simulink model "flight_simulation_6dof"  (R2025b)
settings: Solver=ode4  StartTime=0.0  StopTime=8.6  FixedStep=1/1000  RelTol=1e-3  AbsTol=1e-3  EnableMultiTasking=on
undefined symbols (not defined in the file): X, Y, Z
libraries: nesl_utility x122, sm_lib x98, simulink_extras x48, aerolibatmos2 x4, sharedtransform x4
(part 5 of 6)

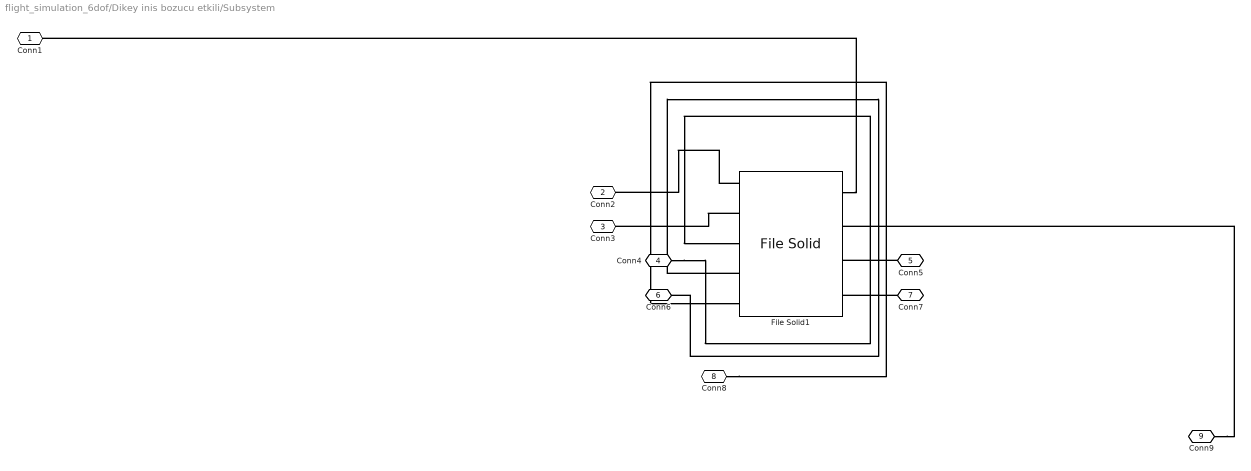
== system flight_simulation_6dof/Dikey inis bozucu etkili/Subsystem ==
  File Solid1 : sm_lib/Body Elements/File Solid  ExtGeomFileName=Roket 2926 Montaj Koordinat Merkeze Alınmış.STEP  UnitType=FromFile  ExtGeomFileUnits=m  StepReaderType=HEX  ExportConvexHullGeometry=off  InertiaType=Custom  BasedOnType=Mass  Density=1000  DensityUnits=kg/m^3  Mass=25  MassUnits=kg  CenterOfMass=[0 0 0.367]  CenterOfMassUnits=m  MomentsOfInertia=[3.842 3.842 1.406]  MomentsOfInertiaUnits=kg*m^2  ProductsOfInertia=[0 0 0]  ProductsOfInertiaUnits=kg*m^2  GraphicType=FromGeometry  MarkerShape=Sphere  MarkerSize=10  GraphicVisPropType=SimpleVisualProperties  GraphicDiffuseColor=[0.5 0.5 0.5]  GraphicOpacity=1  GraphicSpecularColor=[0.5 0.5 0.5 1.0]  GraphicAmbientColor=[0.15 0.15 0.15 1.0]  GraphicEmissiveColor=[0.0 0.0 0.0 1.0]  GraphicShininess=75  DoExposeReferenceFrame=on  SerializedFrames=|
      | <Frames>
      | 
      |   <Frame>
      |     <Id>Frame1</Id>
      |     <Value>
      |       <Name>Nozzle Frame</Name>
      |       <Origin>
      |         <Source>GeometricFeature</Source>
      |         <FeatureName>planar surface 207</FeatureName>
      |       </Origin>
      |       <PrimaryAxis>
      |         <DefinedDirection>+Z</DefinedDirection>
      |         <Source>ReferenceFrame</Source>
      |         <SourceDirection>+Z</SourceDirection>
      |         <FeatureName></FeatureName>
      |       </PrimaryAxis>
      |       <SecondaryAxis>
      |         <DefinedDirection>+X</DefinedDirection>
      |         <Source>ReferenceFrame</Source>
      |         <SourceDirection>+X</SourceDirection>
      |         <FeatureName></FeatureName>
      |       </SecondaryAxis>
      |     </Value>
      |   </Frame>
      | 
      |   <Frame>
      |     <Id>Frame3</Id>
      |     <Value>
      |       <Name>FN</Name>
      |       <Origin>
      |         <Source>GeometricFeature</Source>
      |         <FeatureName>planar surface 225</FeatureName>
      |       </Origin>
      |       <PrimaryAxis>
      |         <DefinedDirection>+Z</DefinedDirection>
      |         <Source>ReferenceFrame</Source>
      |         <SourceDirection>+X</SourceDirection>
      |         <FeatureName></FeatureName>
      |       </PrimaryAxis>
      |       <SecondaryAxis>
      |         <DefinedDirection>+X</DefinedDirection>
      |         <Source>ReferenceFrame</Source>
      |         <SourceDirection>-Z</SourceDirection>
      |         <FeatureName></FeatureName>
      |       </SecondaryAxis>
      |     </Value>
      |   </Frame>
      | 
      |   <Frame>
      |     <Id>Frame2</Id>
      |     <Value>
      |       <Name>Ref_Gas_Container</Name>
      |       <Origin>
      |         <Source>GeometricFeature</Source>
      |         <FeatureName>circular curve 1254</FeatureName>
      |       </Origin>
      |       <PrimaryAxis>
      |         <DefinedDirection>+Z</DefinedDirection>
      |         <Source>ReferenceFrame</Source>
      |         <SourceDirection>+Z</SourceDirection>
      |         <FeatureName></FeatureName>
      |       </PrimaryAxis>
      |       <SecondaryAxis>
      |         <DefinedDirection>+X</DefinedDirection>
      |         <Source>ReferenceFrame</Source>
      |         <SourceDirection>+X</SourceDirection>
      |         <FeatureName></FeatureName>
      |       </SecondaryAxis>
      |     </Value>
      |   </Frame>
      | 
      |   <Frame>
      |     <Id>Frame4</Id>
      |     <Value>
      |       <Name>LL1</Name>
      |       <Origin>
      |         <Source>GeometricFeature</Source>
      |         <FeatureName>circular curve 1452</FeatureName>
      |       </Origin>
      |       <PrimaryAxis>
      |         <DefinedDirection>+Z</DefinedDirection>
      |         <Source>ReferenceFrame</Source>
      |         <SourceDirection>+Z</SourceDirection>
      |         <FeatureName></FeatureName>
      |       </PrimaryAxis>
      |       <SecondaryAxis>
      |         <DefinedDirection>+X</DefinedDirection>
      |         <Source>ReferenceFrame</Source>
      |         <SourceDirection>+X</SourceDirection>
      |         <FeatureName></FeatureName>
      |       </SecondaryAxis>
      |     </Value>
      |   </Frame>
      | 
      |   <Frame>
      |     <Id>Frame5</Id>
      |     <Value>
      |       <Name>LL2</Name>
      |       <Origin>
      |         <Source>GeometricFeature</Source>
      |         <FeatureName>circular curve 188</FeatureName>
      |       </Origin>
      |       <PrimaryAxis>
      |         <DefinedDirection>+Z</DefinedDirection>
      |         <Source>ReferenceFrame</Source>
      |         <SourceDirection>+Z</SourceDirection>
      |         <FeatureName></FeatureName>
      |       </PrimaryAxis>
      |       <SecondaryAxis>
      |         <DefinedDirection>+X</DefinedDirection>
      |         <Source>ReferenceFrame</Source>
      |         <SourceDirection>+X</SourceDirection>
      |         <FeatureName></FeatureName>
      |       </SecondaryAxis>
      |     </Value>
      |   </Frame>
      | 
      |   <Frame>
      |     <Id>Frame6</Id>
      |     <Value>
      |       <Name>LL3</Name>
      |       <Origin>
      |         <Source>GeometricFeature</Source>
      |         <FeatureName>circular curve 1193</FeatureName>
      |       </Origin>
      |       <PrimaryAxis>
      |         <DefinedDirection>+Z</DefinedDirection>
      |         <Source>ReferenceFrame</Source>
      |         <SourceDirection>+Z</SourceDirection>
      |         <FeatureName></FeatureName>
      |       </PrimaryAxis>
      |       <SecondaryAxis>
      |         <DefinedDirection>+X</DefinedDirection>
      |         <Source>ReferenceFrame</Source>
      |         <SourceDirection>+X</SourceDirection>
      |         <FeatureName></FeatureName>
      |       </SecondaryAxis>
      |     </Value>
      |   </Frame>
      | 
      |   <Frame>
      |     <Id>Frame7</Id>
      |     <Value>
      |       <Name>LL4</Name>
      |       <Origin>
      |         <Source>GeometricFeature</Source>
      |         <FeatureName>circular curve 1537</FeatureName>
      |       </Origin>
      |       <PrimaryAxis>
      |         <DefinedDirection>+Z</DefinedDirection>
      |         <Source>ReferenceFrame</Source>
      |         <SourceDirection>+Z</SourceDirection>
      |         <FeatureName></FeatureName>
      |       </PrimaryAxis>
      |       <SecondaryAxis>
      |         <DefinedDirection>+X</DefinedDirection>
      |         <Source>ReferenceFrame</Source>
      |         <SourceDirection>+X</SourceDirection>
      |         <FeatureName></FeatureName>
      |       </SecondaryAxis>
      |     </Value>
      |   </Frame>
      | 
      |   <Frame>
      |     <Id>Frame8</Id>
      |     <Value>
      |       <Name>Dış Kuvvet</Name>
      |       <Origin>
      |         <Source>GeometricFeature</Source>
      |         <FeatureName>cylindrical surface 168</FeatureName>
      |       </Origin>
      |       <PrimaryAxis>
      |         <DefinedDirection>+Z</DefinedDirection>
      |         <Source>ReferenceFrame</Source>
      |         <SourceDirection>+Z</SourceDirection>
      |         <FeatureName></FeatureName>
      |       </PrimaryAxis>
      |       <SecondaryAxis>
      |         <DefinedDirection>+X</DefinedDirection>
      |         <Source>ReferenceFrame</Source>
      |         <SourceDirection>-X</SourceDirection>
      |         <FeatureName></FeatureName>
      |       </SecondaryAxis>
      |     </Value>
      |   </Frame>
      | 
      | </Frames>
  Conn1 : PMIOPort  Side=Right
  Conn2 : PMIOPort  Port=2  Side=Left
  Conn3 : PMIOPort  Port=3  Side=Left
  Conn4 : PMIOPort  Port=4  Side=Left
  Conn5 : PMIOPort  Port=5  Side=Right
  Conn6 : PMIOPort  Port=6  Side=Left
  Conn7 : PMIOPort  Port=7  Side=Right
  Conn8 : PMIOPort  Port=8  Side=Left
  Conn9 : PMIOPort  Port=9  Side=Right
  connections:
  Conn4/RConn1 -- File Solid1/LConn3
  File Solid1/LConn2 -- Conn3/RConn1
  File Solid1/LConn1 -- Conn2/RConn1
  Conn9/RConn1 -- File Solid1/RConn2
  Conn8/RConn1 -- File Solid1/LConn5
  File Solid1/LConn4 -- Conn6/RConn1
  File Solid1/RConn1 -- Conn1/RConn1
  Conn7/RConn1 -- File Solid1/RConn4
  Conn5/RConn1 -- File Solid1/RConn3

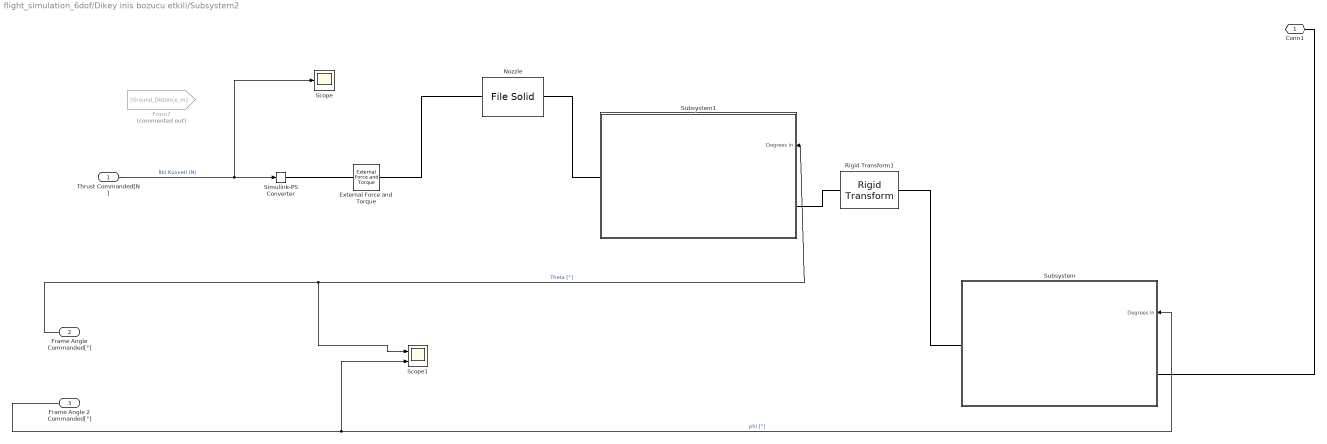
== system flight_simulation_6dof/Dikey inis bozucu etkili/Subsystem2 ==
  Thrust Commanded[N] : Inport
  Frame Angle Commanded[°] : Inport  Port=2
  Frame Angle 2 Commanded[°] : Inport  Port=3
  External Force and Torque : sm_lib/Forces and Torques/External Force and Torque  EnableForceX=off  EnableForceY=off  EnableForceZ=on  EnableForce=off  ForceResolutionFrame=AttachedFrame  EnableTorqueX=off  EnableTorqueY=off  EnableTorqueZ=off  EnableTorque=off  TorqueResolutionFrame=AttachedFrame
  From7 : From  Commented=on  GotoTag=Ground_Distance_m
  Nozzle : sm_lib/Body Elements/File Solid  ExtGeomFileName=C:\Users\HASAN BARAN\Desktop\ucusbenzetimson\S-TEK STEP DOSYALAR\nozzle.STEP  UnitType=FromFile  ExtGeomFileUnits=m  StepReaderType=HEX  ExportConvexHullGeometry=off  InertiaType=Custom  BasedOnType=DensityFromFile  Density=1000  DensityUnits=kg/m^3  Mass=1  MassUnits=kg  CenterOfMass=[0 0 0]  CenterOfMassUnits=m  MomentsOfInertia=[1 1 1]  MomentsOfInertiaUnits=kg*m^2  ProductsOfInertia=[0 0 0]  ProductsOfInertiaUnits=kg*m^2  GraphicType=FromGeometry  MarkerShape=Sphere  MarkerSize=10  GraphicVisPropType=SimpleVisualProperties  GraphicDiffuseColor=[0.5 0.5 0.5]  GraphicOpacity=1  GraphicSpecularColor=[0.5 0.5 0.5 1.0]  GraphicAmbientColor=[0.15 0.15 0.15 1.0]  GraphicEmissiveColor=[0.0 0.0 0.0 1.0]  GraphicShininess=75  DoExposeReferenceFrame=off  SerializedFrames=|
      | <Frames>
      | 
      |   <Frame>
      |     <Id>Frame1</Id>
      |     <Value>
      |       <Name>NF</Name>
      |       <Origin>
      |         <Source>GeometricFeature</Source>
      |         <FeatureName>circular curve 24</FeatureName>
      |       </Origin>
      |       <PrimaryAxis>
      |         <DefinedDirection>+Z</DefinedDirection>
      |         <Source>ReferenceFrame</Source>
      |         <SourceDirection>+X</SourceDirection>
      |         <FeatureName></FeatureName>
      |       </PrimaryAxis>
      |       <SecondaryAxis>
      |         <DefinedDirection>+X</DefinedDirection>
      |         <Source>ReferenceFrame</Source>
      |         <SourceDirection>-Z</SourceDirection>
      |         <FeatureName></FeatureName>
      |       </SecondaryAxis>
      |     </Value>
      |   </Frame>
      | 
      |   <Frame>
      |     <Id>Frame2</Id>
      |     <Value>
      |       <Name>Thrust</Name>
      |       <Origin>
      |         <Source>GeometricFeature</Source>
      |         <FeatureName>planar surface 3</FeatureName>
      |       </Origin>
      |       <PrimaryAxis>
      |         <DefinedDirection>+Z</DefinedDirection>
      |         <Source>ReferenceFrame</Source>
      |         <SourceDirection>+Z</SourceDirection>
      |         <FeatureName></FeatureName>
      |       </PrimaryAxis>
      |       <SecondaryAxis>
      |         <DefinedDirection>+X</DefinedDirection>
      |         <Source>ReferenceFrame</Source>
      |         <SourceDirection>+X</SourceDirection>
      |         <FeatureName></FeatureName>
      |       </SecondaryAxis>
      |     </Value>
      |   </Frame>
      | 
      | </Frames>
  Rigid Transform1 : sm_lib/Frames and Transforms/Rigid Transform  RotationMethod=StandardAxis  FollAlignAxisA=+X  BaseAlignAxisA=+Y  FollAlignAxisB=+Y  BaseAlignAxisB=+Z  RotationStandardAxis=+X  RotationAngle=-90  RotationAngleUnits=deg  RotationArbitraryAxis=[0 0 1]  RotationSequenceAxes=FollowerAxes  RotationSequence=XYX  RotationSequenceAngles=[0 0 0]  RotationSequenceAnglesUnits=deg  RotationMatrix=[1 0 0;0 1 0;0 0 1]  Quaternion=[1 0 0 0]  TranslationMethod=None  TranslationCartesianOffset=[0 0 0]  TranslationCartesianOffsetUnits=m  TranslationStandardAxis=+X  TranslationStandardOffset=0  TranslationStandardOffsetUnits=m  TranslationROffset=0  TranslationROffsetUnits=m  TranslationThetaOffset=0  TranslationThetaOffsetUnits=deg  TranslationZOffset=0  TranslationZOffsetUnits=m
  Scope : Scope
      settings: ActiveDisplayYMinimum=-11.060688029355445  ActiveDisplayYMaximum=24.029985729120519  DataLoggingVariableName=ScopeData6
  Scope1 : Scope  NumInputPorts=2
      settings: ActiveDisplayYMinimum=-79.822032700952221  ActiveDisplayYMaximum=168.51424627565183  DataLoggingVariableName=ScopeData15
  Simulink-PS Converter : nesl_utility/Simulink-PS Converter  PhysicalDomain=network_engine_domain  SubClassName=ps_input  LeftPortType=input  RightPortType=output  PseudoPeriodic=off  Frequencies=[]  NoiseDistribution=none  NoiseParameters=[]  Unit=1  AffineConversion=off  FilteringAndDerivatives=provide  SimscapeFilterOrder=1  InputFilterTimeConstant=0.001  UdotUserProvided=0
  Subsystem : Subsystem
  Subsystem1 : Subsystem
  Conn1 : PMIOPort  Side=Right
  wires:
  Frame Angle 2 Commanded[°]/1 -> Subsystem/1(Degrees in), Scope1/2  "phi [°]"
  Frame Angle Commanded[°]/1 -> Scope1/1, Subsystem1/1(Degrees in)  "Theta [°]"
  Thrust Commanded[N]/1 -> Simulink-PS Converter/1, Scope/1  "İtki Kuvveti (N)"
  connections:
  Simulink-PS Converter/RConn1 -- External Force and Torque/LConn1
  Subsystem/LConn1 -- Conn1/RConn1
  Subsystem/RConn1 -- Rigid Transform1/LConn1
  Rigid Transform1/RConn1 -- Subsystem1/LConn1
  External Force and Torque/RConn1 -- Nozzle/RConn1
  Subsystem1/RConn1 -- Nozzle/LConn1

== system flight_simulation_6dof/Yerden kalkis/MassModel1 ==
  Maximum Mass of Gas [kg] : Constant  Value=5
  Scope : Scope
      settings: ActiveDisplayYMinimum=-0.62488749999999993  ActiveDisplayYMaximum=5.6249875  DataLoggingVariableName=ScopeData11
  m_int : Integrator  InitialConditionSource=external  InitialCondition=31  LimitOutput=on  UpperSaturationLimit=5  LowerSaturationLimit=0.0001
  mdot_cmd : Constant  Commented=on  Value=0.9
  mdot_cmd2 : Step  Time=1.1  After=0.9  SampleTime=0
  negate : Gain  Gain=-1
  Mass of Gas [kg] : Outport
  wires:
  mdot_cmd2/1 -> negate/1
  negate/1 -> m_int/1
  m_int/1 -> Scope/1, Mass of Gas [kg]/1
  Maximum Mass of Gas [kg]/1 -> m_int/2

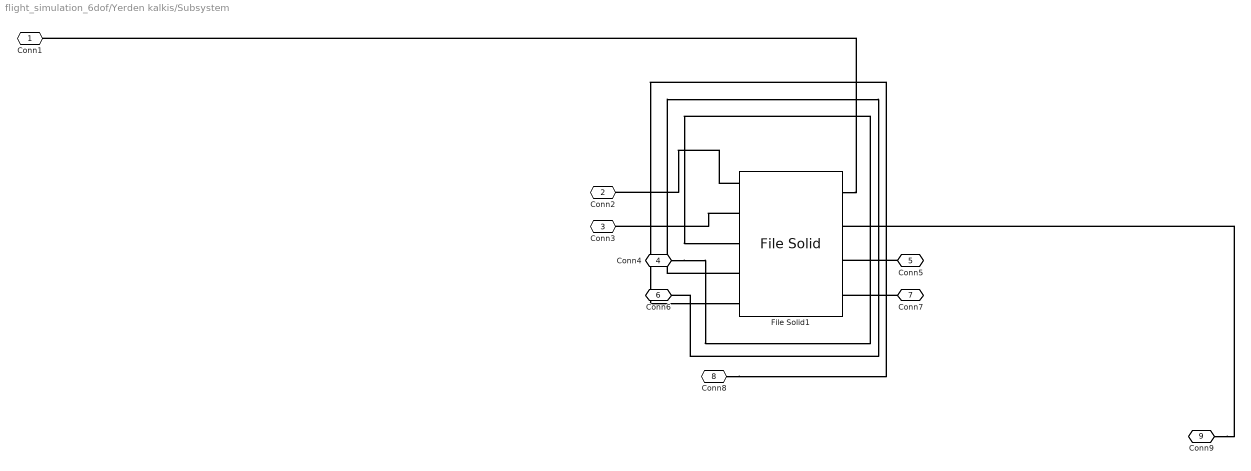
== system flight_simulation_6dof/Yerden kalkis/Subsystem ==
  File Solid1 : sm_lib/Body Elements/File Solid  ExtGeomFileName=Roket 2926 Montaj Koordinat Merkeze Alınmış.STEP  UnitType=FromFile  ExtGeomFileUnits=m  StepReaderType=HEX  ExportConvexHullGeometry=off  InertiaType=Custom  BasedOnType=Mass  Density=1000  DensityUnits=kg/m^3  Mass=25  MassUnits=kg  CenterOfMass=[0 0 0.367]  CenterOfMassUnits=m  MomentsOfInertia=[3.842 3.842 1.406]  MomentsOfInertiaUnits=kg*m^2  ProductsOfInertia=[0 0 0]  ProductsOfInertiaUnits=kg*m^2  GraphicType=FromGeometry  MarkerShape=Sphere  MarkerSize=10  GraphicVisPropType=SimpleVisualProperties  GraphicDiffuseColor=[0.5 0.5 0.5]  GraphicOpacity=1  GraphicSpecularColor=[0.5 0.5 0.5 1.0]  GraphicAmbientColor=[0.15 0.15 0.15 1.0]  GraphicEmissiveColor=[0.0 0.0 0.0 1.0]  GraphicShininess=75  DoExposeReferenceFrame=on  SerializedFrames=|
      | <Frames>
      | 
      |   <Frame>
      |     <Id>Frame1</Id>
      |     <Value>
      |       <Name>Nozzle Frame</Name>
      |       <Origin>
      |         <Source>GeometricFeature</Source>
      |         <FeatureName>planar surface 207</FeatureName>
      |       </Origin>
      |       <PrimaryAxis>
      |         <DefinedDirection>+Z</DefinedDirection>
      |         <Source>ReferenceFrame</Source>
      |         <SourceDirection>+Z</SourceDirection>
      |         <FeatureName></FeatureName>
      |       </PrimaryAxis>
      |       <SecondaryAxis>
      |         <DefinedDirection>+X</DefinedDirection>
      |         <Source>ReferenceFrame</Source>
      |         <SourceDirection>+X</SourceDirection>
      |         <FeatureName></FeatureName>
      |       </SecondaryAxis>
      |     </Value>
      |   </Frame>
      | 
      |   <Frame>
      |     <Id>Frame3</Id>
      |     <Value>
      |       <Name>FN</Name>
      |       <Origin>
      |         <Source>GeometricFeature</Source>
      |         <FeatureName>planar surface 225</FeatureName>
      |       </Origin>
      |       <PrimaryAxis>
      |         <DefinedDirection>+Z</DefinedDirection>
      |         <Source>ReferenceFrame</Source>
      |         <SourceDirection>+X</SourceDirection>
      |         <FeatureName></FeatureName>
      |       </PrimaryAxis>
      |       <SecondaryAxis>
      |         <DefinedDirection>+X</DefinedDirection>
      |         <Source>ReferenceFrame</Source>
      |         <SourceDirection>-Z</SourceDirection>
      |         <FeatureName></FeatureName>
      |       </SecondaryAxis>
      |     </Value>
      |   </Frame>
      | 
      |   <Frame>
      |     <Id>Frame2</Id>
      |     <Value>
      |       <Name>Ref_Gas_Container</Name>
      |       <Origin>
      |         <Source>GeometricFeature</Source>
      |         <FeatureName>circular curve 1254</FeatureName>
      |       </Origin>
      |       <PrimaryAxis>
      |         <DefinedDirection>+Z</DefinedDirection>
      |         <Source>ReferenceFrame</Source>
      |         <SourceDirection>+Z</SourceDirection>
      |         <FeatureName></FeatureName>
      |       </PrimaryAxis>
      |       <SecondaryAxis>
      |         <DefinedDirection>+X</DefinedDirection>
      |         <Source>ReferenceFrame</Source>
      |         <SourceDirection>+X</SourceDirection>
      |         <FeatureName></FeatureName>
      |       </SecondaryAxis>
      |     </Value>
      |   </Frame>
      | 
      |   <Frame>
      |     <Id>Frame4</Id>
      |     <Value>
      |       <Name>LL1</Name>
      |       <Origin>
      |         <Source>GeometricFeature</Source>
      |         <FeatureName>circular curve 1452</FeatureName>
      |       </Origin>
      |       <PrimaryAxis>
      |         <DefinedDirection>+Z</DefinedDirection>
      |         <Source>ReferenceFrame</Source>
      |         <SourceDirection>+Z</SourceDirection>
      |         <FeatureName></FeatureName>
      |       </PrimaryAxis>
      |       <SecondaryAxis>
      |         <DefinedDirection>+X</DefinedDirection>
      |         <Source>ReferenceFrame</Source>
      |         <SourceDirection>+X</SourceDirection>
      |         <FeatureName></FeatureName>
      |       </SecondaryAxis>
      |     </Value>
      |   </Frame>
      | 
      |   <Frame>
      |     <Id>Frame5</Id>
      |     <Value>
      |       <Name>LL2</Name>
      |       <Origin>
      |         <Source>GeometricFeature</Source>
      |         <FeatureName>circular curve 188</FeatureName>
      |       </Origin>
      |       <PrimaryAxis>
      |         <DefinedDirection>+Z</DefinedDirection>
      |         <Source>ReferenceFrame</Source>
      |         <SourceDirection>+Z</SourceDirection>
      |         <FeatureName></FeatureName>
      |       </PrimaryAxis>
      |       <SecondaryAxis>
      |         <DefinedDirection>+X</DefinedDirection>
      |         <Source>ReferenceFrame</Source>
      |         <SourceDirection>+X</SourceDirection>
      |         <FeatureName></FeatureName>
      |       </SecondaryAxis>
      |     </Value>
      |   </Frame>
      | 
      |   <Frame>
      |     <Id>Frame6</Id>
      |     <Value>
      |       <Name>LL3</Name>
      |       <Origin>
      |         <Source>GeometricFeature</Source>
      |         <FeatureName>circular curve 1193</FeatureName>
      |       </Origin>
      |       <PrimaryAxis>
      |         <DefinedDirection>+Z</DefinedDirection>
      |         <Source>ReferenceFrame</Source>
      |         <SourceDirection>+Z</SourceDirection>
      |         <FeatureName></FeatureName>
      |       </PrimaryAxis>
      |       <SecondaryAxis>
      |         <DefinedDirection>+X</DefinedDirection>
      |         <Source>ReferenceFrame</Source>
      |         <SourceDirection>+X</SourceDirection>
      |         <FeatureName></FeatureName>
      |       </SecondaryAxis>
      |     </Value>
      |   </Frame>
      | 
      |   <Frame>
      |     <Id>Frame7</Id>
      |     <Value>
      |       <Name>LL4</Name>
      |       <Origin>
      |         <Source>GeometricFeature</Source>
      |         <FeatureName>circular curve 1537</FeatureName>
      |       </Origin>
      |       <PrimaryAxis>
      |         <DefinedDirection>+Z</DefinedDirection>
      |         <Source>ReferenceFrame</Source>
      |         <SourceDirection>+Z</SourceDirection>
      |         <FeatureName></FeatureName>
      |       </PrimaryAxis>
      |       <SecondaryAxis>
      |         <DefinedDirection>+X</DefinedDirection>
      |         <Source>ReferenceFrame</Source>
      |         <SourceDirection>+X</SourceDirection>
      |         <FeatureName></FeatureName>
      |       </SecondaryAxis>
      |     </Value>
      |   </Frame>
      | 
      |   <Frame>
      |     <Id>Frame8</Id>
      |     <Value>
      |       <Name>Dış Kuvvet</Name>
      |       <Origin>
      |         <Source>GeometricFeature</Source>
      |         <FeatureName>cylindrical surface 168</FeatureName>
      |       </Origin>
      |       <PrimaryAxis>
      |         <DefinedDirection>+Z</DefinedDirection>
      |         <Source>ReferenceFrame</Source>
      |         <SourceDirection>+Z</SourceDirection>
      |         <FeatureName></FeatureName>
      |       </PrimaryAxis>
      |       <SecondaryAxis>
      |         <DefinedDirection>+X</DefinedDirection>
      |         <Source>ReferenceFrame</Source>
      |         <SourceDirection>-X</SourceDirection>
      |         <FeatureName></FeatureName>
      |       </SecondaryAxis>
      |     </Value>
      |   </Frame>
      | 
      | </Frames>
  Conn1 : PMIOPort  Side=Right
  Conn2 : PMIOPort  Port=2  Side=Left
  Conn3 : PMIOPort  Port=3  Side=Left
  Conn4 : PMIOPort  Port=4  Side=Left
  Conn5 : PMIOPort  Port=5  Side=Right
  Conn6 : PMIOPort  Port=6  Side=Left
  Conn7 : PMIOPort  Port=7  Side=Right
  Conn8 : PMIOPort  Port=8  Side=Left
  Conn9 : PMIOPort  Port=9  Side=Right
  connections:
  Conn5/RConn1 -- File Solid1/RConn3
  Conn7/RConn1 -- File Solid1/RConn4
  File Solid1/RConn1 -- Conn1/RConn1
  File Solid1/LConn4 -- Conn6/RConn1
  Conn8/RConn1 -- File Solid1/LConn5
  Conn9/RConn1 -- File Solid1/RConn2
  File Solid1/LConn1 -- Conn2/RConn1
  File Solid1/LConn2 -- Conn3/RConn1
  Conn4/RConn1 -- File Solid1/LConn3

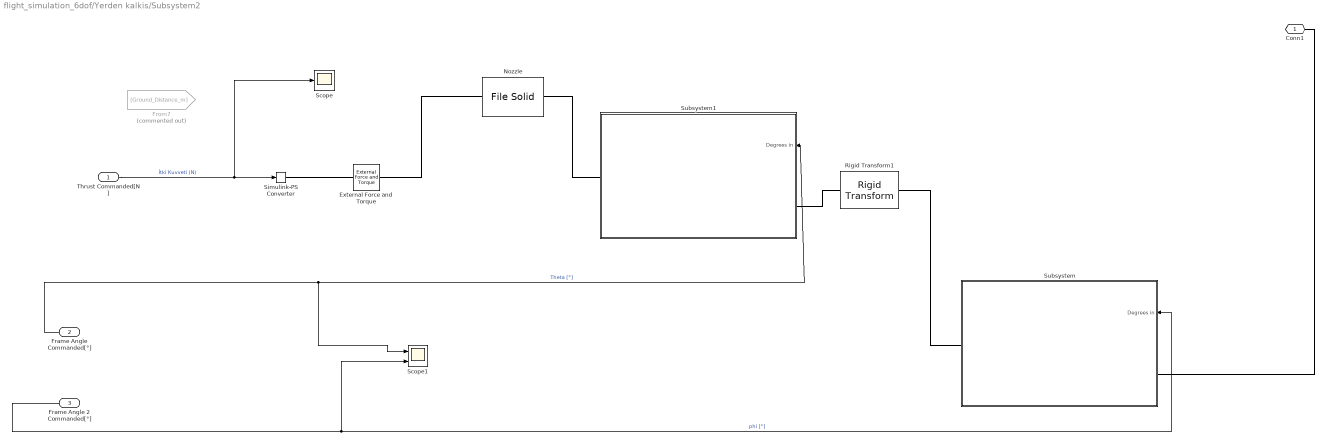
== system flight_simulation_6dof/Yerden kalkis/Subsystem2 ==
  Thrust Commanded[N] : Inport
  Frame Angle Commanded[°] : Inport  Port=2
  Frame Angle 2 Commanded[°] : Inport  Port=3
  External Force and Torque : sm_lib/Forces and Torques/External Force and Torque  EnableForceX=off  EnableForceY=off  EnableForceZ=on  EnableForce=off  ForceResolutionFrame=AttachedFrame  EnableTorqueX=off  EnableTorqueY=off  EnableTorqueZ=off  EnableTorque=off  TorqueResolutionFrame=AttachedFrame
  From7 : From  Commented=on  GotoTag=Ground_Distance_m
  Nozzle : sm_lib/Body Elements/File Solid  ExtGeomFileName=C:\Users\HASAN BARAN\Desktop\ucusbenzetimson\S-TEK STEP DOSYALAR\nozzle.STEP  UnitType=FromFile  ExtGeomFileUnits=m  StepReaderType=HEX  ExportConvexHullGeometry=off  InertiaType=Custom  BasedOnType=DensityFromFile  Density=1000  DensityUnits=kg/m^3  Mass=1  MassUnits=kg  CenterOfMass=[0 0 0]  CenterOfMassUnits=m  MomentsOfInertia=[1 1 1]  MomentsOfInertiaUnits=kg*m^2  ProductsOfInertia=[0 0 0]  ProductsOfInertiaUnits=kg*m^2  GraphicType=FromGeometry  MarkerShape=Sphere  MarkerSize=10  GraphicVisPropType=SimpleVisualProperties  GraphicDiffuseColor=[0.5 0.5 0.5]  GraphicOpacity=1  GraphicSpecularColor=[0.5 0.5 0.5 1.0]  GraphicAmbientColor=[0.15 0.15 0.15 1.0]  GraphicEmissiveColor=[0.0 0.0 0.0 1.0]  GraphicShininess=75  DoExposeReferenceFrame=off  SerializedFrames=|
      | <Frames>
      | 
      |   <Frame>
      |     <Id>Frame1</Id>
      |     <Value>
      |       <Name>NF</Name>
      |       <Origin>
      |         <Source>GeometricFeature</Source>
      |         <FeatureName>circular curve 24</FeatureName>
      |       </Origin>
      |       <PrimaryAxis>
      |         <DefinedDirection>+Z</DefinedDirection>
      |         <Source>ReferenceFrame</Source>
      |         <SourceDirection>+X</SourceDirection>
      |         <FeatureName></FeatureName>
      |       </PrimaryAxis>
      |       <SecondaryAxis>
      |         <DefinedDirection>+X</DefinedDirection>
      |         <Source>ReferenceFrame</Source>
      |         <SourceDirection>-Z</SourceDirection>
      |         <FeatureName></FeatureName>
      |       </SecondaryAxis>
      |     </Value>
      |   </Frame>
      | 
      |   <Frame>
      |     <Id>Frame2</Id>
      |     <Value>
      |       <Name>Thrust</Name>
      |       <Origin>
      |         <Source>GeometricFeature</Source>
      |         <FeatureName>planar surface 3</FeatureName>
      |       </Origin>
      |       <PrimaryAxis>
      |         <DefinedDirection>+Z</DefinedDirection>
      |         <Source>ReferenceFrame</Source>
      |         <SourceDirection>+Z</SourceDirection>
      |         <FeatureName></FeatureName>
      |       </PrimaryAxis>
      |       <SecondaryAxis>
      |         <DefinedDirection>+X</DefinedDirection>
      |         <Source>ReferenceFrame</Source>
      |         <SourceDirection>+X</SourceDirection>
      |         <FeatureName></FeatureName>
      |       </SecondaryAxis>
      |     </Value>
      |   </Frame>
      | 
      | </Frames>
  Rigid Transform1 : sm_lib/Frames and Transforms/Rigid Transform  RotationMethod=StandardAxis  FollAlignAxisA=+X  BaseAlignAxisA=+Y  FollAlignAxisB=+Y  BaseAlignAxisB=+Z  RotationStandardAxis=+X  RotationAngle=-90  RotationAngleUnits=deg  RotationArbitraryAxis=[0 0 1]  RotationSequenceAxes=FollowerAxes  RotationSequence=XYX  RotationSequenceAngles=[0 0 0]  RotationSequenceAnglesUnits=deg  RotationMatrix=[1 0 0;0 1 0;0 0 1]  Quaternion=[1 0 0 0]  TranslationMethod=None  TranslationCartesianOffset=[0 0 0]  TranslationCartesianOffsetUnits=m  TranslationStandardAxis=+X  TranslationStandardOffset=0  TranslationStandardOffsetUnits=m  TranslationROffset=0  TranslationROffsetUnits=m  TranslationThetaOffset=0  TranslationThetaOffsetUnits=deg  TranslationZOffset=0  TranslationZOffsetUnits=m
  Scope : Scope
      settings: ActiveDisplayYMinimum=-11.060688029355445  ActiveDisplayYMaximum=24.029985729120519  DataLoggingVariableName=ScopeData6
  Scope1 : Scope  NumInputPorts=2
      settings: ActiveDisplayYMinimum=-79.822032700952221  ActiveDisplayYMaximum=168.51424627565183  DataLoggingVariableName=ScopeData15
  Simulink-PS Converter : nesl_utility/Simulink-PS Converter  PhysicalDomain=network_engine_domain  SubClassName=ps_input  LeftPortType=input  RightPortType=output  PseudoPeriodic=off  Frequencies=[]  NoiseDistribution=none  NoiseParameters=[]  Unit=1  AffineConversion=off  FilteringAndDerivatives=provide  SimscapeFilterOrder=1  InputFilterTimeConstant=0.001  UdotUserProvided=0
  Subsystem : Subsystem
  Subsystem1 : Subsystem
  Conn1 : PMIOPort  Side=Right
  wires:
  Thrust Commanded[N]/1 -> Scope/1, Simulink-PS Converter/1  "İtki Kuvveti (N)"
  Frame Angle Commanded[°]/1 -> Subsystem1/1(Degrees in), Scope1/1  "Theta [°]"
  Frame Angle 2 Commanded[°]/1 -> Scope1/2, Subsystem/1(Degrees in)  "phi [°]"
  connections:
  Subsystem1/RConn1 -- Nozzle/LConn1
  External Force and Torque/RConn1 -- Nozzle/RConn1
  Rigid Transform1/RConn1 -- Subsystem1/LConn1
  Subsystem/RConn1 -- Rigid Transform1/LConn1
  Subsystem/LConn1 -- Conn1/RConn1
  Simulink-PS Converter/RConn1 -- External Force and Torque/LConn1

== system flight_simulation_6dof/Yerden kalkis bozucu etkili/MassModel1 ==
  Maximum Mass of Gas [kg] : Constant  Value=5
  Scope : Scope
      settings: ActiveDisplayYMinimum=-0.62488749999999993  ActiveDisplayYMaximum=5.6249875  DataLoggingVariableName=ScopeData11
  m_int : Integrator  InitialConditionSource=external  InitialCondition=31  LimitOutput=on  UpperSaturationLimit=5  LowerSaturationLimit=0.0001
  mdot_cmd : Constant  Commented=on  Value=0.9
  mdot_cmd2 : Step  Time=1.1  After=0.9  SampleTime=0
  negate : Gain  Gain=-1
  Mass of Gas [kg] : Outport
  wires:
  Maximum Mass of Gas [kg]/1 -> m_int/2
  m_int/1 -> Mass of Gas [kg]/1, Scope/1
  negate/1 -> m_int/1
  mdot_cmd2/1 -> negate/1

== system flight_simulation_6dof/Yerden kalkis bozucu etkili/Subsystem ==
  File Solid1 : sm_lib/Body Elements/File Solid  ExtGeomFileName=Roket 2926 Montaj Koordinat Merkeze Alınmış.STEP  UnitType=FromFile  ExtGeomFileUnits=m  StepReaderType=HEX  ExportConvexHullGeometry=off  InertiaType=Custom  BasedOnType=Mass  Density=1000  DensityUnits=kg/m^3  Mass=25  MassUnits=kg  CenterOfMass=[0 0 0.367]  CenterOfMassUnits=m  MomentsOfInertia=[3.842 3.842 1.406]  MomentsOfInertiaUnits=kg*m^2  ProductsOfInertia=[0 0 0]  ProductsOfInertiaUnits=kg*m^2  GraphicType=FromGeometry  MarkerShape=Sphere  MarkerSize=10  GraphicVisPropType=SimpleVisualProperties  GraphicDiffuseColor=[0.5 0.5 0.5]  GraphicOpacity=1  GraphicSpecularColor=[0.5 0.5 0.5 1.0]  GraphicAmbientColor=[0.15 0.15 0.15 1.0]  GraphicEmissiveColor=[0.0 0.0 0.0 1.0]  GraphicShininess=75  DoExposeReferenceFrame=on  SerializedFrames=|
      | <Frames>
      | 
      |   <Frame>
      |     <Id>Frame1</Id>
      |     <Value>
      |       <Name>Nozzle Frame</Name>
      |       <Origin>
      |         <Source>GeometricFeature</Source>
      |         <FeatureName>planar surface 207</FeatureName>
      |       </Origin>
      |       <PrimaryAxis>
      |         <DefinedDirection>+Z</DefinedDirection>
      |         <Source>ReferenceFrame</Source>
      |         <SourceDirection>+Z</SourceDirection>
      |         <FeatureName></FeatureName>
      |       </PrimaryAxis>
      |       <SecondaryAxis>
      |         <DefinedDirection>+X</DefinedDirection>
      |         <Source>ReferenceFrame</Source>
      |         <SourceDirection>+X</SourceDirection>
      |         <FeatureName></FeatureName>
      |       </SecondaryAxis>
      |     </Value>
      |   </Frame>
      | 
      |   <Frame>
      |     <Id>Frame3</Id>
      |     <Value>
      |       <Name>FN</Name>
      |       <Origin>
      |         <Source>GeometricFeature</Source>
      |         <FeatureName>planar surface 225</FeatureName>
      |       </Origin>
      |       <PrimaryAxis>
      |         <DefinedDirection>+Z</DefinedDirection>
      |         <Source>ReferenceFrame</Source>
      |         <SourceDirection>+X</SourceDirection>
      |         <FeatureName></FeatureName>
      |       </PrimaryAxis>
      |       <SecondaryAxis>
      |         <DefinedDirection>+X</DefinedDirection>
      |         <Source>ReferenceFrame</Source>
      |         <SourceDirection>-Z</SourceDirection>
      |         <FeatureName></FeatureName>
      |       </SecondaryAxis>
      |     </Value>
      |   </Frame>
      | 
      |   <Frame>
      |     <Id>Frame2</Id>
      |     <Value>
      |       <Name>Ref_Gas_Container</Name>
      |       <Origin>
      |         <Source>GeometricFeature</Source>
      |         <FeatureName>circular curve 1254</FeatureName>
      |       </Origin>
      |       <PrimaryAxis>
      |         <DefinedDirection>+Z</DefinedDirection>
      |         <Source>ReferenceFrame</Source>
      |         <SourceDirection>+Z</SourceDirection>
      |         <FeatureName></FeatureName>
      |       </PrimaryAxis>
      |       <SecondaryAxis>
      |         <DefinedDirection>+X</DefinedDirection>
      |         <Source>ReferenceFrame</Source>
      |         <SourceDirection>+X</SourceDirection>
      |         <FeatureName></FeatureName>
      |       </SecondaryAxis>
      |     </Value>
      |   </Frame>
      | 
      |   <Frame>
      |     <Id>Frame4</Id>
      |     <Value>
      |       <Name>LL1</Name>
      |       <Origin>
      |         <Source>GeometricFeature</Source>
      |         <FeatureName>circular curve 1452</FeatureName>
      |       </Origin>
      |       <PrimaryAxis>
      |         <DefinedDirection>+Z</DefinedDirection>
      |         <Source>ReferenceFrame</Source>
      |         <SourceDirection>+Z</SourceDirection>
      |         <FeatureName></FeatureName>
      |       </PrimaryAxis>
      |       <SecondaryAxis>
      |         <DefinedDirection>+X</DefinedDirection>
      |         <Source>ReferenceFrame</Source>
      |         <SourceDirection>+X</SourceDirection>
      |         <FeatureName></FeatureName>
      |       </SecondaryAxis>
      |     </Value>
      |   </Frame>
      | 
      |   <Frame>
      |     <Id>Frame5</Id>
      |     <Value>
      |       <Name>LL2</Name>
      |       <Origin>
      |         <Source>GeometricFeature</Source>
      |         <FeatureName>circular curve 188</FeatureName>
      |       </Origin>
      |       <PrimaryAxis>
      |         <DefinedDirection>+Z</DefinedDirection>
      |         <Source>ReferenceFrame</Source>
      |         <SourceDirection>+Z</SourceDirection>
      |         <FeatureName></FeatureName>
      |       </PrimaryAxis>
      |       <SecondaryAxis>
      |         <DefinedDirection>+X</DefinedDirection>
      |         <Source>ReferenceFrame</Source>
      |         <SourceDirection>+X</SourceDirection>
      |         <FeatureName></FeatureName>
      |       </SecondaryAxis>
      |     </Value>
      |   </Frame>
      | 
      |   <Frame>
      |     <Id>Frame6</Id>
      |     <Value>
      |       <Name>LL3</Name>
      |       <Origin>
      |         <Source>GeometricFeature</Source>
      |         <FeatureName>circular curve 1193</FeatureName>
      |       </Origin>
      |       <PrimaryAxis>
      |         <DefinedDirection>+Z</DefinedDirection>
      |         <Source>ReferenceFrame</Source>
      |         <SourceDirection>+Z</SourceDirection>
      |         <FeatureName></FeatureName>
      |       </PrimaryAxis>
      |       <SecondaryAxis>
      |         <DefinedDirection>+X</DefinedDirection>
      |         <Source>ReferenceFrame</Source>
      |         <SourceDirection>+X</SourceDirection>
      |         <FeatureName></FeatureName>
      |       </SecondaryAxis>
      |     </Value>
      |   </Frame>
      | 
      |   <Frame>
      |     <Id>Frame7</Id>
      |     <Value>
      |       <Name>LL4</Name>
      |       <Origin>
      |         <Source>GeometricFeature</Source>
      |         <FeatureName>circular curve 1537</FeatureName>
      |       </Origin>
      |       <PrimaryAxis>
      |         <DefinedDirection>+Z</DefinedDirection>
      |         <Source>ReferenceFrame</Source>
      |         <SourceDirection>+Z</SourceDirection>
      |         <FeatureName></FeatureName>
      |       </PrimaryAxis>
      |       <SecondaryAxis>
      |         <DefinedDirection>+X</DefinedDirection>
      |         <Source>ReferenceFrame</Source>
      |         <SourceDirection>+X</SourceDirection>
      |         <FeatureName></FeatureName>
      |       </SecondaryAxis>
      |     </Value>
      |   </Frame>
      | 
      |   <Frame>
      |     <Id>Frame8</Id>
      |     <Value>
      |       <Name>Dış Kuvvet</Name>
      |       <Origin>
      |         <Source>GeometricFeature</Source>
      |         <FeatureName>cylindrical surface 168</FeatureName>
      |       </Origin>
      |       <PrimaryAxis>
      |         <DefinedDirection>+Z</DefinedDirection>
      |         <Source>ReferenceFrame</Source>
      |         <SourceDirection>+Z</SourceDirection>
      |         <FeatureName></FeatureName>
      |       </PrimaryAxis>
      |       <SecondaryAxis>
      |         <DefinedDirection>+X</DefinedDirection>
      |         <Source>ReferenceFrame</Source>
      |         <SourceDirection>-X</SourceDirection>
      |         <FeatureName></FeatureName>
      |       </SecondaryAxis>
      |     </Value>
      |   </Frame>
      | 
      | </Frames>
  Conn1 : PMIOPort  Side=Right
  Conn2 : PMIOPort  Port=2  Side=Left
  Conn3 : PMIOPort  Port=3  Side=Left
  Conn4 : PMIOPort  Port=4  Side=Left
  Conn5 : PMIOPort  Port=5  Side=Right
  Conn6 : PMIOPort  Port=6  Side=Left
  Conn7 : PMIOPort  Port=7  Side=Right
  Conn8 : PMIOPort  Port=8  Side=Left
  Conn9 : PMIOPort  Port=9  Side=Right
  connections:
  Conn4/RConn1 -- File Solid1/LConn3
  File Solid1/LConn2 -- Conn3/RConn1
  File Solid1/LConn1 -- Conn2/RConn1
  Conn9/RConn1 -- File Solid1/RConn2
  Conn8/RConn1 -- File Solid1/LConn5
  File Solid1/LConn4 -- Conn6/RConn1
  File Solid1/RConn1 -- Conn1/RConn1
  Conn7/RConn1 -- File Solid1/RConn4
  Conn5/RConn1 -- File Solid1/RConn3

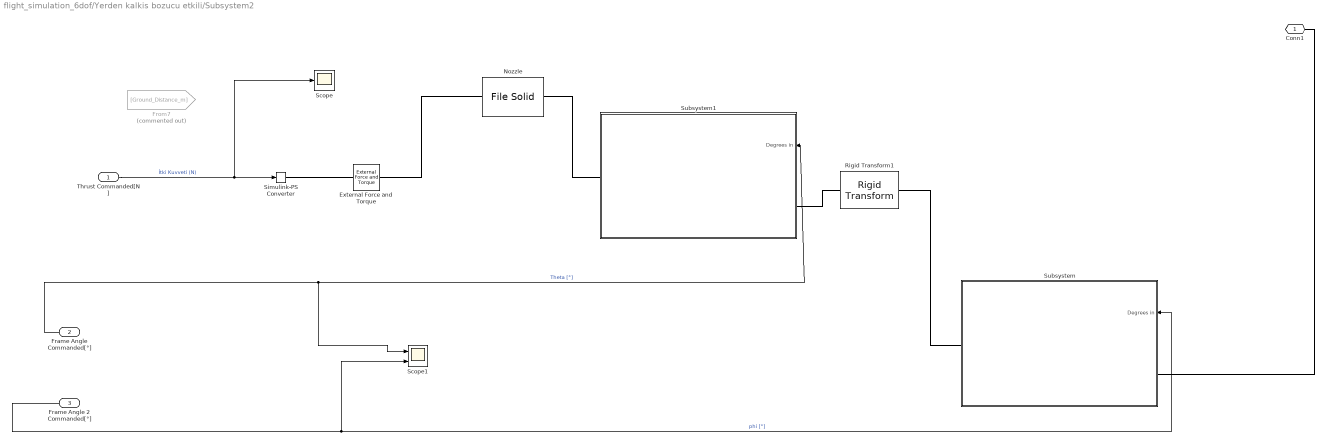
== system flight_simulation_6dof/Yerden kalkis bozucu etkili/Subsystem2 ==
  Thrust Commanded[N] : Inport
  Frame Angle Commanded[°] : Inport  Port=2
  Frame Angle 2 Commanded[°] : Inport  Port=3
  External Force and Torque : sm_lib/Forces and Torques/External Force and Torque  EnableForceX=off  EnableForceY=off  EnableForceZ=on  EnableForce=off  ForceResolutionFrame=AttachedFrame  EnableTorqueX=off  EnableTorqueY=off  EnableTorqueZ=off  EnableTorque=off  TorqueResolutionFrame=AttachedFrame
  From7 : From  Commented=on  GotoTag=Ground_Distance_m
  Nozzle : sm_lib/Body Elements/File Solid  ExtGeomFileName=C:\Users\HASAN BARAN\Desktop\ucusbenzetimson\S-TEK STEP DOSYALAR\nozzle.STEP  UnitType=FromFile  ExtGeomFileUnits=m  StepReaderType=HEX  ExportConvexHullGeometry=off  InertiaType=Custom  BasedOnType=DensityFromFile  Density=1000  DensityUnits=kg/m^3  Mass=1  MassUnits=kg  CenterOfMass=[0 0 0]  CenterOfMassUnits=m  MomentsOfInertia=[1 1 1]  MomentsOfInertiaUnits=kg*m^2  ProductsOfInertia=[0 0 0]  ProductsOfInertiaUnits=kg*m^2  GraphicType=FromGeometry  MarkerShape=Sphere  MarkerSize=10  GraphicVisPropType=SimpleVisualProperties  GraphicDiffuseColor=[0.5 0.5 0.5]  GraphicOpacity=1  GraphicSpecularColor=[0.5 0.5 0.5 1.0]  GraphicAmbientColor=[0.15 0.15 0.15 1.0]  GraphicEmissiveColor=[0.0 0.0 0.0 1.0]  GraphicShininess=75  DoExposeReferenceFrame=off  SerializedFrames=|
      | <Frames>
      | 
      |   <Frame>
      |     <Id>Frame1</Id>
      |     <Value>
      |       <Name>NF</Name>
      |       <Origin>
      |         <Source>GeometricFeature</Source>
      |         <FeatureName>circular curve 24</FeatureName>
      |       </Origin>
      |       <PrimaryAxis>
      |         <DefinedDirection>+Z</DefinedDirection>
      |         <Source>ReferenceFrame</Source>
      |         <SourceDirection>+X</SourceDirection>
      |         <FeatureName></FeatureName>
      |       </PrimaryAxis>
      |       <SecondaryAxis>
      |         <DefinedDirection>+X</DefinedDirection>
      |         <Source>ReferenceFrame</Source>
      |         <SourceDirection>-Z</SourceDirection>
      |         <FeatureName></FeatureName>
      |       </SecondaryAxis>
      |     </Value>
      |   </Frame>
      | 
      |   <Frame>
      |     <Id>Frame2</Id>
      |     <Value>
      |       <Name>Thrust</Name>
      |       <Origin>
      |         <Source>GeometricFeature</Source>
      |         <FeatureName>planar surface 3</FeatureName>
      |       </Origin>
      |       <PrimaryAxis>
      |         <DefinedDirection>+Z</DefinedDirection>
      |         <Source>ReferenceFrame</Source>
      |         <SourceDirection>+Z</SourceDirection>
      |         <FeatureName></FeatureName>
      |       </PrimaryAxis>
      |       <SecondaryAxis>
      |         <DefinedDirection>+X</DefinedDirection>
      |         <Source>ReferenceFrame</Source>
      |         <SourceDirection>+X</SourceDirection>
      |         <FeatureName></FeatureName>
      |       </SecondaryAxis>
      |     </Value>
      |   </Frame>
      | 
      | </Frames>
  Rigid Transform1 : sm_lib/Frames and Transforms/Rigid Transform  RotationMethod=StandardAxis  FollAlignAxisA=+X  BaseAlignAxisA=+Y  FollAlignAxisB=+Y  BaseAlignAxisB=+Z  RotationStandardAxis=+X  RotationAngle=-90  RotationAngleUnits=deg  RotationArbitraryAxis=[0 0 1]  RotationSequenceAxes=FollowerAxes  RotationSequence=XYX  RotationSequenceAngles=[0 0 0]  RotationSequenceAnglesUnits=deg  RotationMatrix=[1 0 0;0 1 0;0 0 1]  Quaternion=[1 0 0 0]  TranslationMethod=None  TranslationCartesianOffset=[0 0 0]  TranslationCartesianOffsetUnits=m  TranslationStandardAxis=+X  TranslationStandardOffset=0  TranslationStandardOffsetUnits=m  TranslationROffset=0  TranslationROffsetUnits=m  TranslationThetaOffset=0  TranslationThetaOffsetUnits=deg  TranslationZOffset=0  TranslationZOffsetUnits=m
  Scope : Scope
      settings: ActiveDisplayYMinimum=-11.060688029355445  ActiveDisplayYMaximum=24.029985729120519  DataLoggingVariableName=ScopeData6
  Scope1 : Scope  NumInputPorts=2
      settings: ActiveDisplayYMinimum=-79.822032700952221  ActiveDisplayYMaximum=168.51424627565183  DataLoggingVariableName=ScopeData15
  Simulink-PS Converter : nesl_utility/Simulink-PS Converter  PhysicalDomain=network_engine_domain  SubClassName=ps_input  LeftPortType=input  RightPortType=output  PseudoPeriodic=off  Frequencies=[]  NoiseDistribution=none  NoiseParameters=[]  Unit=1  AffineConversion=off  FilteringAndDerivatives=provide  SimscapeFilterOrder=1  InputFilterTimeConstant=0.001  UdotUserProvided=0
  Subsystem : Subsystem
  Subsystem1 : Subsystem
  Conn1 : PMIOPort  Side=Right
  wires:
  Frame Angle 2 Commanded[°]/1 -> Subsystem/1(Degrees in), Scope1/2  "phi [°]"
  Frame Angle Commanded[°]/1 -> Scope1/1, Subsystem1/1(Degrees in)  "Theta [°]"
  Thrust Commanded[N]/1 -> Simulink-PS Converter/1, Scope/1  "İtki Kuvveti (N)"
  connections:
  Simulink-PS Converter/RConn1 -- External Force and Torque/LConn1
  Subsystem/LConn1 -- Conn1/RConn1
  Subsystem/RConn1 -- Rigid Transform1/LConn1
  Rigid Transform1/RConn1 -- Subsystem1/LConn1
  External Force and Torque/RConn1 -- Nozzle/RConn1
  Subsystem1/RConn1 -- Nozzle/LConn1

== system flight_simulation_6dof/Dikey inis/Subsystem2/Subsystem ==
  Degrees in : Inport
  Constant1 : Constant  Value=0
  Constant2 : Constant  Value=0
  Degrees to Radians : simulink_extras/Transformations/Degrees to Radians
  Rate Limiter : RateLimiter  RisingSlewLimit=deg2rad(12)/0.3  FallingSlewLimit=-deg2rad(12)/0.3  SampleTimeMode=inherited
  Revolute Joint : sm_lib/Joints/Revolute Joint  JointMode=Normal  CompositeWrenchDir=FollowerOnBase  CompositeWrenchFrame=BaseFrame  SenseConstraintForce=off  SenseConstraintTorque=off  SenseTotalForce=off  SenseTotalTorque=off  PositionTargetSpecify=off  PositionTargetPriority=High  PositionTargetValue=0  PositionTargetValueUnits=deg  VelocityTargetSpecify=off  VelocityTargetPriority=High  VelocityTargetValue=0  VelocityTargetValueUnits=deg/s  EquilibriumPosition=0  EquilibriumPositionUnits=deg  SpringStiffness=0  SpringStiffnessUnits=N*m/deg  DampingCoefficient=0  DampingCoefficientUnits=N*m/(deg/s)  LowerLimitSpecify=off  LowerLimitBound=-90  LowerLimitBoundUnits=deg  LowerLimitStiffness=1e4  LowerLimitStiffnessUnits=N*m/deg  LowerLimitDamping=10  LowerLimitDampingUnits=N*m/(deg/s)  LowerLimitTransitionRegionWidth=0.1  LowerLimitTransitionRegionWidthUnits=deg  UpperLimitSpecify=off  UpperLimitBound=90  UpperLimitBoundUnits=deg  UpperLimitStiffness=1e4  UpperLimitStiffnessUnits=N*m/deg  UpperLimitDamping=10  UpperLimitDampingUnits=N*m/(deg/s)  UpperLimitTransitionRegionWidth=0.1  UpperLimitTransitionRegionWidthUnits=deg  TorqueActuationMode=ComputedTorque  MotionActuationMode=InputMotion  SensePosition=off  SenseVelocity=off  SenseAcceleration=off  SenseTorqueForce=off  SenseLowerLimitTorqueForce=off  SenseUpperLimitTorqueForce=off
  Simulink-PS Converter : nesl_utility/Simulink-PS Converter  PhysicalDomain=network_engine_domain  SubClassName=ps_input  LeftPortType=input  RightPortType=output  PseudoPeriodic=off  Frequencies=[]  NoiseDistribution=none  NoiseParameters=[]  Unit=1  AffineConversion=off  FilteringAndDerivatives=provide  SimscapeFilterOrder=1  InputFilterTimeConstant=0.001  UdotUserProvided=2
  Conn1 : PMIOPort  Side=Left
  Conn2 : PMIOPort  Port=2  Side=Right
  wires:
  Degrees in/1 -> Degrees to Radians/1
  Constant2/1 -> Simulink-PS Converter/3
  Constant1/1 -> Simulink-PS Converter/2
  Degrees to Radians/1 -> Rate Limiter/1
  Rate Limiter/1 -> Simulink-PS Converter/1
  connections:
  Simulink-PS Converter/RConn1 -- Revolute Joint/LConn2
  Revolute Joint/RConn1 -- Conn2/RConn1
  Revolute Joint/LConn1 -- Conn1/RConn1

== system flight_simulation_6dof/Dikey inis/Subsystem2/Subsystem1 ==
  Degrees in : Inport
  Constant : Constant  Value=0
  Constant1 : Constant  Value=0
  Degrees to Radians : simulink_extras/Transformations/Degrees to Radians
  Rate Limiter : RateLimiter  RisingSlewLimit=deg2rad(12)/0.3  FallingSlewLimit=-deg2rad(12)/0.3  SampleTimeMode=inherited
  Revolute Joint : sm_lib/Joints/Revolute Joint  JointMode=Normal  CompositeWrenchDir=FollowerOnBase  CompositeWrenchFrame=BaseFrame  SenseConstraintForce=off  SenseConstraintTorque=off  SenseTotalForce=off  SenseTotalTorque=off  PositionTargetSpecify=off  PositionTargetPriority=High  PositionTargetValue=0  PositionTargetValueUnits=deg  VelocityTargetSpecify=off  VelocityTargetPriority=High  VelocityTargetValue=0  VelocityTargetValueUnits=deg/s  EquilibriumPosition=0  EquilibriumPositionUnits=deg  SpringStiffness=0  SpringStiffnessUnits=N*m/deg  DampingCoefficient=0  DampingCoefficientUnits=N*m/(deg/s)  LowerLimitSpecify=off  LowerLimitBound=-90  LowerLimitBoundUnits=deg  LowerLimitStiffness=1e4  LowerLimitStiffnessUnits=N*m/deg  LowerLimitDamping=10  LowerLimitDampingUnits=N*m/(deg/s)  LowerLimitTransitionRegionWidth=0.1  LowerLimitTransitionRegionWidthUnits=deg  UpperLimitSpecify=off  UpperLimitBound=90  UpperLimitBoundUnits=deg  UpperLimitStiffness=1e4  UpperLimitStiffnessUnits=N*m/deg  UpperLimitDamping=10  UpperLimitDampingUnits=N*m/(deg/s)  UpperLimitTransitionRegionWidth=0.1  UpperLimitTransitionRegionWidthUnits=deg  TorqueActuationMode=ComputedTorque  MotionActuationMode=InputMotion  SensePosition=off  SenseVelocity=off  SenseAcceleration=off  SenseTorqueForce=off  SenseLowerLimitTorqueForce=off  SenseUpperLimitTorqueForce=off
  Simulink-PS Converter : nesl_utility/Simulink-PS Converter  PhysicalDomain=network_engine_domain  SubClassName=ps_input  LeftPortType=input  RightPortType=output  PseudoPeriodic=off  Frequencies=[]  NoiseDistribution=none  NoiseParameters=[]  Unit=1  AffineConversion=off  FilteringAndDerivatives=provide  SimscapeFilterOrder=1  InputFilterTimeConstant=0.001  UdotUserProvided=2
  Conn1 : PMIOPort  Side=Left
  Conn2 : PMIOPort  Port=2  Side=Right
  wires:
  Degrees in/1 -> Degrees to Radians/1
  Degrees to Radians/1 -> Rate Limiter/1
  Constant/1 -> Simulink-PS Converter/2
  Constant1/1 -> Simulink-PS Converter/3
  Rate Limiter/1 -> Simulink-PS Converter/1
  connections:
  Revolute Joint/LConn1 -- Conn1/RConn1
  Revolute Joint/RConn1 -- Conn2/RConn1
  Simulink-PS Converter/RConn1 -- Revolute Joint/LConn2

== system flight_simulation_6dof/Dikey inis bozucu etkili/Subsystem2/Subsystem ==
  Degrees in : Inport
  Constant1 : Constant  Value=0
  Constant2 : Constant  Value=0
  Degrees to Radians : simulink_extras/Transformations/Degrees to Radians
  Rate Limiter : RateLimiter  RisingSlewLimit=deg2rad(12)/0.3  FallingSlewLimit=-deg2rad(12)/0.3  SampleTimeMode=inherited
  Revolute Joint : sm_lib/Joints/Revolute Joint  JointMode=Normal  CompositeWrenchDir=FollowerOnBase  CompositeWrenchFrame=BaseFrame  SenseConstraintForce=off  SenseConstraintTorque=off  SenseTotalForce=off  SenseTotalTorque=off  PositionTargetSpecify=off  PositionTargetPriority=High  PositionTargetValue=0  PositionTargetValueUnits=deg  VelocityTargetSpecify=off  VelocityTargetPriority=High  VelocityTargetValue=0  VelocityTargetValueUnits=deg/s  EquilibriumPosition=0  EquilibriumPositionUnits=deg  SpringStiffness=0  SpringStiffnessUnits=N*m/deg  DampingCoefficient=0  DampingCoefficientUnits=N*m/(deg/s)  LowerLimitSpecify=off  LowerLimitBound=-90  LowerLimitBoundUnits=deg  LowerLimitStiffness=1e4  LowerLimitStiffnessUnits=N*m/deg  LowerLimitDamping=10  LowerLimitDampingUnits=N*m/(deg/s)  LowerLimitTransitionRegionWidth=0.1  LowerLimitTransitionRegionWidthUnits=deg  UpperLimitSpecify=off  UpperLimitBound=90  UpperLimitBoundUnits=deg  UpperLimitStiffness=1e4  UpperLimitStiffnessUnits=N*m/deg  UpperLimitDamping=10  UpperLimitDampingUnits=N*m/(deg/s)  UpperLimitTransitionRegionWidth=0.1  UpperLimitTransitionRegionWidthUnits=deg  TorqueActuationMode=ComputedTorque  MotionActuationMode=InputMotion  SensePosition=off  SenseVelocity=off  SenseAcceleration=off  SenseTorqueForce=off  SenseLowerLimitTorqueForce=off  SenseUpperLimitTorqueForce=off
  Simulink-PS Converter : nesl_utility/Simulink-PS Converter  PhysicalDomain=network_engine_domain  SubClassName=ps_input  LeftPortType=input  RightPortType=output  PseudoPeriodic=off  Frequencies=[]  NoiseDistribution=none  NoiseParameters=[]  Unit=1  AffineConversion=off  FilteringAndDerivatives=provide  SimscapeFilterOrder=1  InputFilterTimeConstant=0.001  UdotUserProvided=2
  Conn1 : PMIOPort  Side=Left
  Conn2 : PMIOPort  Port=2  Side=Right
  wires:
  Rate Limiter/1 -> Simulink-PS Converter/1
  Degrees to Radians/1 -> Rate Limiter/1
  Constant1/1 -> Simulink-PS Converter/2
  Constant2/1 -> Simulink-PS Converter/3
  Degrees in/1 -> Degrees to Radians/1
  connections:
  Revolute Joint/LConn1 -- Conn1/RConn1
  Revolute Joint/RConn1 -- Conn2/RConn1
  Simulink-PS Converter/RConn1 -- Revolute Joint/LConn2
